simulink model "hydro_simulink_model"  (R2026b)
settings: Solver=VariableStepAuto
libraries: fuzblock x1
settings Model: Creator=Popescu  LastModifiedBy=Popescu

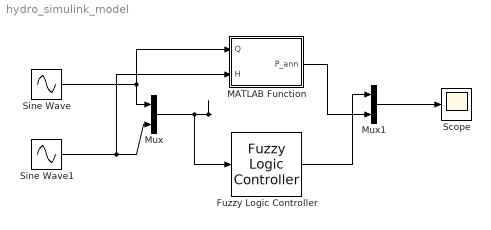
== system hydro_simulink_model ==
  Fuzzy Logic Controller : fuzblock/Fuzzy Logic  Controller  FIS='hydro_fuzzy_controller.fis'  OutputSampleNumber=101  DataType=double  UseLookupTable=off  NumBreakpoints=10  FuzzifiedInputs=off  RuleFiringStrengths=off  RuleOutputs=off  AggregatedOutputs=off  SimulateUsing=Interpreted execution  OutOfRangeInputValueMessage=warning  NoRuleFiredMessage=warning  EmptyOutputFuzzySetMessage=warning
  MATLAB Function : MATLAB Function  TreatAsAtomicUnit=on
  Mux : Mux  Inputs=2
  Mux1 : Mux  Inputs=2
  Scope : Scope
      settings: ActiveDisplayYMinimum=-4.2788802517901274  ActiveDisplayYMaximum=118.98483862924689
  Sine Wave : Sin  Amplitude=100  Bias=115  SampleTime=0
  Sine Wave1 : Sin  Amplitude=20  Bias=42.5  Frequency=0.5  SampleTime=0
  wires:
  Sine Wave/1 -> MATLAB Function/1(Q), Mux/1
  Sine Wave1/1 -> MATLAB Function/2(H), Mux/2
  Mux/1 -> Fuzzy Logic Controller/1
  MATLAB Function/1(P_ann) -> Mux1/2
  Fuzzy Logic Controller/1 -> Mux1/1
  Mux1/1 -> Scope/1

== matlab function hydro_simulink_model/MATLAB Function ==
  data: Q input; P_ann output; H input
function P_ann = fcn(Q, H)
P_ann = 0;
persistent net
if isempty(net)
    net = loadLearnerForCoder('trained_ann_model.mat')
end
pred = predict(net, [double(Q), double(H)]);
P_ann = double(pred(1));
end
